simulink library "Linkage_Decoupled_Link5"  (R2026a)
settings: Solver=VariableStepAuto
undefined symbols (not defined in the file): Init, Left, Linkage, Visual, X, Y, Z
libraries: sm_lib x56, Suspension_Utilities x23, fl_lib x1, nesl_utility x1
(part 1 of 3)
Description:
  | Component of Simscape Vehicle Templates Library
  | 
  | Copyright 2018-2024 The MathWorks, Inc.
settings Model: Creator=smiller  LastModifiedBy=andrei

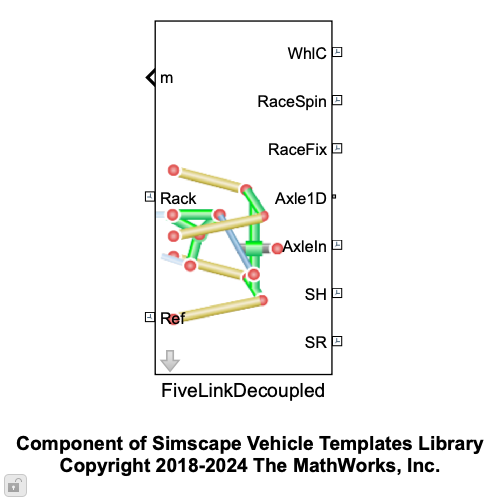
[thumbnail: Simulink's stored preview of the top-level diagram]
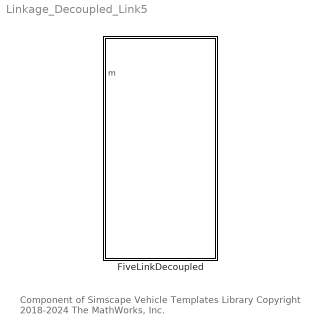
== system Linkage_Decoupled_Link5 ==
  note: Component of Simscape Vehicle Templates Library
      | Copyright 2018-2024 The MathWorks, Inc.
  FiveLinkDecoupled : Subsystem  VariantControl=FiveLinkShockFront  mask(Five-Link Suspension, Decoupled){popup_leftRight=Left, hp_in_f_ua=Linkage.UpperArmF.sInboard.Value, hp_in_r_ua=Linkage.UpperArmR.sInboard.Value, hp_out_f_ua=Linkage.UpperArmF.sOutboard.Value, hp_out_r_ua=Linkage.UpperArmR.sOutboard.Value, hp_in_f_la=Linkage.LowerArmF.sInboard.Value, hp_in_r_la=Linkage.LowerArmR.sInboard.Value, hp_out_f_la=Linkage.LowerArmF.sOutboard.Value, hp_out_r_la=Linkage.LowerArmR.sOutboard.Value, hp_pushrod_in=Linkage.Pushrod.sBellcrank.Value, hp_pushrod_out=Linkage.Pushrod.sUpright.Value, hp_bcr_pivot=Linkage.Bellcrank.sPivot.Value, hp_bcr_shock_heaveL=Linkage.Shock.sHeaveL.Value, hp_bcr_shock_heaveR=Linkage.Shock.sHeaveR.Value, hp_bcr_shock_rollL=Linkage.Shock.sRollL.Value, hp_bcr_shock_rollR=Linkage.Shock.sRollR.Value, hp_upr_cg=Linkage.Upright.sCG.Value, hp_upr_wc=Linkage.Upright.sWheelCentre.Value, hp_in_rod=Linkage.TrackRod.sInboard.Value, hp_upr_rod=Linkage.TrackRod.sOutboard.Value, clr_hp=Visual.hp.clr, opc_hp=Visual.hp.opc, size_hp=Visual.hp.rad, UpperArmF_to_Subframe=Linkage.UpperArmF_to_Subframe, UpperArmR_to_Subframe=Linkage.UpperArmR_to_Subframe, LowerArmF_to_Subframe=Linkage.LowerArmF_to_Subframe, LowerArmR_to_Subframe=Linkage.LowerArmR_to_Subframe, uaf_mass=Linkage.UpperArmF.m.Value, uar_mass=Linkage.UpperArmR.m.Value, laf_mass=Linkage.LowerArmF.m.Value, lar_mass=Linkage.LowerArmR.m.Value, clr_conn_links=Visual.hp.clr, opc_conn_links=Visual.hp.opc, size_conn_links=Visual.hp.rad, clr_uaf=Visual.UpperArm.clr, opc_uaf=Visual.part.opc, radius_uaf=Visual.UpperArm.rad, clr_uar=Visual.UpperArm.clr, opc_uar=Visual.part.opc, radius_uar=Visual.UpperArm.rad, clr_laf=Visual.LowerArm.clr, opc_laf=Visual.part.opc, radius_laf=Visual.LowerArm.rad, clr_lar=Visual.LowerArm.clr, opc_lar=Visual.part.opc, radius_lar=Visual.LowerArm.rad, atoe=Linkage.Upright.aToe.Value, acamber=Linkage.Upright.aCamber.Value, upr_mass=Linkage.Upright.m.Value, axle_len=Linkage.Upright.xAxle.Value, axle_whlc_to_bearing=Linkage.Upright.xWCtoBearing.Value, axle_mass=Linkage.Upright.mAxle.Value, clr_conn_upr=Visual.hp.clr, opc_conn_upr=Visual.hp.opc, size_conn_upr=Visual.hp.rad, clr_upr=Visual.Upright.clr, opc_upr=Visual.part.opc, radius_upr=Visual.Upright.rad, clr_axle=Visual.Axle.clr, opc_axle=Visual.part.opc, radius_axle=Visual.Axle.rad, rod_mass=Linkage.TrackRod.m.Value, clr_conn_rod=Visual.hp.clr, opc_conn_rod=Visual.hp.opc, size_conn_rod=Visual.hp.rad, clr_rod=Visual.TrackRod.clr, opc_rod=Visual.part.opc, radius_rod=Visual.TrackRod.rad, bcr_mass=Linkage.Bellcrank.m.Value, clr_bcr=Visual.Bellcrank.clr, opc_bcr=Visual.part.opc, radius_bcr=Visual.Bellcrank.rad, pushrod_mass=Linkage.Pushrod.m.Value, clr_conn_pushrod=Visual.hp.clr, opc_conn_pushrod=Visual.hp.opc, size_conn_pushrod=Visual.hp.rad, clr_pushrod=Visual.Pushrod.clr, opc_pushrod=Visual.part.opc, radius_pushrod=Visual.Pushrod.rad, whl_init_spd_lr=Init.nWheel.Value}
      mask prompts: popup_leftRight "Left/Right"; hp_in_f_ua "Upper Arm Front [xyz] (m)"; hp_in_r_ua "Upper Arm Rear [xyz] (m)"; hp_out_f_ua "Upper Arm Front Outboard [xyz] (m)"; hp_out_r_ua "Upper Arm Rear Outboard [xyz] (m)"; hp_in_f_la "Lower Arm Front [xyz] (m)"; hp_in_r_la "Lower Arm Rear [xyz] (m)"; hp_out_f_la "Lower Arm Front Outboard [xyz] (m)"; hp_out_r_la "Lower Arm Rear Outboard [xyz] (m)"; hp_pushrod_in "Pushrod Bellcrank [xyz] (m)"; hp_pushrod_out "Pushrod Upright [xyz] (m)"; hp_bcr_pivot "Bellcrank Pivot [xyz] (m)"; hp_bcr_shock_heaveL "Bellcrank Shock Heave Left [xyz] (m)"; hp_bcr_shock_heaveR "Bellcrank Shock Heave Right [xyz] (m)"; hp_bcr_shock_rollL "Bellcrank Shock Roll Left [xyz] (m)"; hp_bcr_shock_rollR "Bellcrank Shock Roll Right [xyz] (m)"; hp_upr_cg "Upright CG [xyz] (m)"; hp_upr_wc "Wheel Center [xyz] (m)"; hp_in_rod "Track Rod Inboard [xyz] (m)"; hp_upr_rod "Track Rod Outboard [xyz] (m)"; atoe "Toe Angle (deg)"; acamber "Camber Angle (deg)"; upr_mass "Mass (kg)"; axle_len "Axle Length (m)"; axle_whlc_to_bearing "Distance Wheel Ctr to Bearing (m)"; axle_mass "Axle Mass (kg)"; rod_mass "Mass (kg)"; bcr_mass "Mass (kg)"; pushrod_mass "Mass (kg)"; whl_init_spd_lr "Initial Wheel Speed (rad/s)"
      mask help: Models a multi-link, decoupled suspension with two upper and two lower control arms connecting the subframe to the upright. Mechanical connections via a bellcrank permit this design to decouple stiffness and damping for body roll and heave.
      mask init:
      | if(popup_leftRight == 1)
      |     rhs_susp = 1;
      |     %whlind = 1;
      |     whl_init_spd = whl_init_spd_lr(1);
      |     hp_bcr_shock_heave = hp_bcr_shock_heaveL;
      |     hp_bcr_shock_roll = hp_bcr_shock_rollL;
      | elseif(popup_leftRight == 2)
      |     rhs_susp = -1;
      |     %whlind = 2;
      | 	whl_init_spd = whl_init_spd_lr(2);
      |     hp_bcr_shock_heave = hp_bcr_shock_heaveR;
      |     hp_bcr_shock_roll = hp_bcr_shock_rollR;    
      | end
      mask TypeOptions popup_leftRight:
      | Hardpoints/popup_leftRight | Upright/popup_leftRight | Lower Arm Rear/popup_leftRight | Lower Arm Front/popup_leftRight | Track Rod/popup_leftRight | Upper Arm Front/popup_leftRight | Upper Arm Rear/popup_leftRight | Universal
      | HP LAF/popup_leftRight | Universal
      | HP LAR/popup_leftRight | Universal
      | HP UAF/popup_leftRight | Universal
      | HP UAR/popup_leftRight | Pushrod/popup_leftRight | Bellcrank/popup_leftRight | HP Bellcrank/popup_leftRight
      mask TypeOptions hp_in_f_ua:
      | Hardpoints/hp_in_f_ua | Universal
      | HP UAF/hp_joint | Upper Arm Front/hp_in
      mask TypeOptions hp_in_r_ua:
      | Hardpoints/hp_in_r_ua | Universal
      | HP UAR/hp_joint | Upper Arm Rear/hp_in
      mask TypeOptions hp_out_f_ua: Upper Arm Front/hp_out | Upright/hp_uaf_out
      mask TypeOptions hp_out_r_ua: Upper Arm Rear/hp_out | Upright/hp_uar_out
      mask TypeOptions hp_in_f_la:
      | Hardpoints/hp_in_f_la | Lower Arm Front/hp_in | Universal
      | HP LAF/hp_joint
      mask TypeOptions hp_in_r_la:
      | Hardpoints/hp_in_r_la | Lower Arm Rear/hp_in | Universal
      | HP LAR/hp_joint
      mask TypeOptions hp_out_f_la: Upright/hp_laf_out | Lower Arm Front/hp_out
      mask TypeOptions hp_out_r_la: Upright/hp_lar_out | Lower Arm Rear/hp_out
      mask TypeOptions hp_pushrod_in: Pushrod/hp_in | Bellcrank/hp_pushrod | HP Bellcrank/hp_pushrod_in
      mask TypeOptions hp_pushrod_out: Pushrod/hp_out | Upright/hp_pushrod
      mask TypeOptions hp_bcr_pivot: Bellcrank/hp_bcr_pivot | HP Bellcrank/hp_bcr_pivot | Hardpoints/hp_bellcrank
      mask TypeOptions hp_upr_cg: Upright/hp_upr_cg
      mask TypeOptions hp_upr_wc: Upright/hp_upr_wc
      mask TypeOptions hp_in_rod: Track Rod/hp_in
      mask TypeOptions hp_upr_rod: Track Rod/hp_out | Upright/hp_upr_rod
      mask TypeOptions clr_hp: Hardpoints/clr_hp
      mask TypeOptions opc_hp: Hardpoints/opc_hp
      mask TypeOptions size_hp: Hardpoints/size_hp
      mask TypeOptions uaf_mass: Upper Arm Front/rod_mass
      mask TypeOptions uar_mass: Upper Arm Rear/rod_mass
      mask TypeOptions laf_mass: Lower Arm Front/rod_mass
      mask TypeOptions lar_mass: Lower Arm Rear/rod_mass
      mask TypeOptions clr_conn_links: Upper Arm Front/clr_conn_rod | Upper Arm Rear/clr_conn_rod | Lower Arm Front/clr_conn_rod | Lower Arm Rear/clr_conn_rod
      mask TypeOptions opc_conn_links: Upper Arm Front/opc_conn_rod | Upper Arm Rear/opc_conn_rod | Lower Arm Front/opc_conn_rod | Lower Arm Rear/opc_conn_rod
      mask TypeOptions size_conn_links: Upper Arm Front/size_conn_rod | Upper Arm Rear/size_conn_rod | Lower Arm Front/size_conn_rod | Lower Arm Rear/size_conn_rod
      mask TypeOptions clr_uaf: Upper Arm Front/clr_rod
      mask TypeOptions opc_uaf: Upper Arm Front/opc_rod
      mask TypeOptions radius_uaf: Upper Arm Front/radius_rod
      mask TypeOptions clr_uar: Upper Arm Rear/clr_rod
      mask TypeOptions opc_uar: Upper Arm Rear/opc_rod
      mask TypeOptions radius_uar: Upper Arm Rear/radius_rod
      mask TypeOptions clr_laf: Lower Arm Front/clr_rod
      mask TypeOptions opc_laf: Lower Arm Front/opc_rod
      mask TypeOptions radius_laf: Lower Arm Front/radius_rod
      mask TypeOptions clr_lar: Lower Arm Rear/clr_rod
      mask TypeOptions opc_lar: Lower Arm Rear/opc_rod
      mask TypeOptions radius_lar: Lower Arm Rear/radius_rod
      mask TypeOptions atoe: Upright/atoe
      mask TypeOptions acamber: Upright/acamber
      mask TypeOptions upr_mass: Upright/upr_mass
      mask TypeOptions axle_len: Upright/axle_len
      mask TypeOptions axle_whlc_to_bearing: Upright/axle_whlc_to_bearing
      mask TypeOptions axle_mass: Upright/axle_mass
      mask TypeOptions clr_conn_upr: Upright/clr_conn_upr
      mask TypeOptions opc_conn_upr: Upright/opc_conn_upr
      mask TypeOptions size_conn_upr: Upright/size_conn_upr
      mask TypeOptions clr_upr: Upright/clr_upr
      mask TypeOptions opc_upr: Upright/opc_upr
      mask TypeOptions radius_upr: Upright/radius_upr
      mask TypeOptions clr_axle: Upright/clr_axle
      mask TypeOptions opc_axle: Upright/opc_axle
      mask TypeOptions radius_axle: Upright/radius_axle
      mask TypeOptions rod_mass: Track Rod/rod_mass
      mask TypeOptions clr_conn_rod: Track Rod/clr_conn_rod
      mask TypeOptions opc_conn_rod: Track Rod/opc_conn_rod
      mask TypeOptions size_conn_rod: Track Rod/size_conn_rod
      mask TypeOptions clr_rod: Track Rod/clr_rod
      mask TypeOptions opc_rod: Track Rod/opc_rod
      mask TypeOptions radius_rod: Track Rod/radius_rod
      mask TypeOptions bcr_mass: Bellcrank/bcr_mass
      mask TypeOptions clr_bcr: Bellcrank/clr_bcr
      mask TypeOptions opc_bcr: Bellcrank/opc_bcr
      mask TypeOptions radius_bcr: Bellcrank/radius_bcr
      mask TypeOptions pushrod_mass: Pushrod/rod_mass
      mask TypeOptions clr_conn_pushrod: Pushrod/clr_conn_rod
      mask TypeOptions opc_conn_pushrod: Pushrod/opc_conn_rod
      mask TypeOptions size_conn_pushrod: Pushrod/size_conn_rod
      mask TypeOptions clr_pushrod: Pushrod/clr_rod
      mask TypeOptions opc_pushrod: Pushrod/opc_rod
      mask TypeOptions radius_pushrod: Pushrod/radius_rod
      mask DialogControl cont_hp Prompt: Hardpoints
      mask DialogControl cont_vis_hp Prompt: Visualization
      mask DialogControl text_clr_hp Prompt: Color [RGB]
      mask DialogControl text_opc_hp Prompt: Opac. (0-1)
      mask DialogControl text_size_hp Prompt: Size (m)
      mask DialogControl text_hp Prompt: Hardpoints
      mask DialogControl cont_links Prompt: Links
      mask DialogControl text_links_part_subf Prompt: Part
      mask DialogControl text_links_subf Prompt: Subframe Connection
      mask DialogControl text_upper_f_subf Prompt: Upper, Front
      mask DialogControl text_upper_r_subf Prompt: Upper, Rear
      mask DialogControl text_lower_f_subf Prompt: Lower, Front
      mask DialogControl text_lower_r_subf Prompt: Lower, Rear
      mask DialogControl text_links_part Prompt: Part
      mask DialogControl text_links_mass Prompt: Mass (kg)
      mask DialogControl text_upper_f Prompt: Upper, Front
      mask DialogControl text_upper_r Prompt: Upper, Rear
      mask DialogControl text_lower_f Prompt: Lower, Front
      mask DialogControl text_lower_r Prompt: Lower, Rear
      mask DialogControl cont_vis_links Prompt: Visualization
      mask DialogControl text_vis_links_clr Prompt: Color [RGB]
      mask DialogControl text_vis_links_opc Prompt: Opacity (0-1)
      mask DialogControl text_vis_links_rad Prompt: Radius (m)
      mask DialogControl text_vis_links_conn Prompt: Connections
      mask DialogControl text_vis_links_uaf Prompt: Upper, Front
      mask DialogControl text_vis_links_uar Prompt: Upper, Rear
      mask DialogControl text_vis_links_laf Prompt: Lower, Front
      mask DialogControl text_vis_links_lar Prompt: Lower, Rear
      mask DialogControl cont_upright Prompt: Upright
      mask DialogControl grp_upright Prompt: Upright
      mask DialogControl grp_upright_axle Prompt: Axle
      mask DialogControl cont_vis_upr Prompt: Visualization
      mask DialogControl text_clr_upr Prompt: Color [RGB]
      mask DialogControl text_opc_upr Prompt: Opac. (0-1)
      mask DialogControl text_size_upr Prompt: Size (m)
      mask DialogControl text_conn_upr Prompt: Connections
      mask DialogControl text_upright Prompt: Upright
      mask DialogControl text_axle Prompt: Axle
      mask DialogControl cont_steer Prompt: Steer
      mask DialogControl grp_rod Prompt: Rod
      mask DialogControl cont_vis_rod Prompt: Visualization
      mask DialogControl text_clr_rod Prompt: Color [RGB]
      mask DialogControl text_opc_rod Prompt: Opac. (0-1)
      mask DialogControl text_size_rod Prompt: Size (m)
      mask DialogControl text_conn_rod Prompt: Connections
      mask DialogControl text_rod_rod Prompt: Rod
      mask DialogControl cont_bellcrank Prompt: Bellcrank
      mask DialogControl grp_bellcrank Prompt: Bellcrank
      mask DialogControl cont_vis_bellcrank Prompt: Visualization
      mask DialogControl text_clr_bellcrank Prompt: Color [RGB]
      mask DialogControl text_opc_bellcrank Prompt: Opac. (0-1)
      mask DialogControl text_size_bellcrank Prompt: Size (m)
      mask DialogControl text_bellcrank Prompt: Bellcrank
      mask DialogControl cont_push Prompt: Pushrod
      mask DialogControl grp_pushrod Prompt: Pushrod
      mask DialogControl cont_vis_pushrod Prompt: Visualization
      mask DialogControl text_clr_pushrod Prompt: Color [RGB]
      mask DialogControl text_opc_pushrod Prompt: Opac. (0-1)
      mask DialogControl text_size_pushrod Prompt: Size (m)
      mask DialogControl text_conn_pushrod Prompt: Connections
      mask DialogControl text_pushrod Prompt: Pushrod
      mask DialogControl cont_initial Prompt: Initial
      mask Display: image('sm_car_vehicle_linkage_5ldec_IMAGE.png');
